simulink subsystem "Vision_Field_Errors_sub"  (R2023b)
settings: Solver=VariableStepAuto  StartTime=0.0  StopTime=10.0  RelTol=1e-3
undefined symbols (not defined in the file): AT_Cage_L_Finish_Angle_Blue, AT_Cage_L_Finish_Angle_Red, AT_Cage_L_Finish_X_Blue, AT_Cage_L_Finish_X_Red, AT_Cage_L_Finish_Y_Blue, AT_Cage_L_Finish_Y_Red, AT_Cage_L_Start_Angle_Blue, AT_Cage_L_Start_Angle_Red, AT_Cage_L_Start_X_Blue, AT_Cage_L_Start_X_Red, AT_Cage_L_Start_Y_Blue, AT_Cage_L_Start_Y_Red, AT_Cage_M_Finish_Angle_Blue, AT_Cage_M_Finish_Angle_Red, AT_Cage_M_Finish_X_Blue, AT_Cage_M_Finish_X_Red, AT_Cage_M_Finish_Y_Blue, AT_Cage_M_Finish_Y_Red, AT_Cage_M_Start_Angle_Blue, AT_Cage_M_Start_Angle_Red, AT_Cage_M_Start_X_Blue, AT_Cage_M_Start_X_Red, AT_Cage_M_Start_Y_Blue, AT_Cage_M_Start_Y_Red, AT_Cage_R_Finish_Angle_Blue, AT_Cage_R_Finish_Angle_Red, AT_Cage_R_Finish_X_Blue, AT_Cage_R_Finish_X_Red, AT_Cage_R_Finish_Y_Blue, AT_Cage_R_Finish_Y_Red, AT_Cage_R_Start_Angle_Blue, AT_Cage_R_Start_Angle_Red, AT_Cage_R_Start_X_Blue, AT_Cage_R_Start_X_Red, AT_Cage_R_Start_Y_Blue, AT_Cage_R_Start_Y_Red, AT_CS_L_Angle_Blue, AT_CS_L_Angle_Red, AT_CS_L_X_Blue, AT_CS_L_X_Red, AT_CS_L_Y_Blue, AT_CS_L_Y_Red, AT_CS_R_Angle_Blue, AT_CS_R_Angle_Red, AT_CS_R_X_Blue, AT_CS_R_X_Red, AT_CS_R_Y_Blue, AT_CS_R_Y_Red, AT_Processor_Angle_Blue, AT_Processor_Angle_Red, AT_Processor_X_Blue, AT_Processor_X_Red, AT_Processor_Y_Blue, AT_Processor_Y_Red
settings Model: Creator=ander  LastModifiedBy=ander

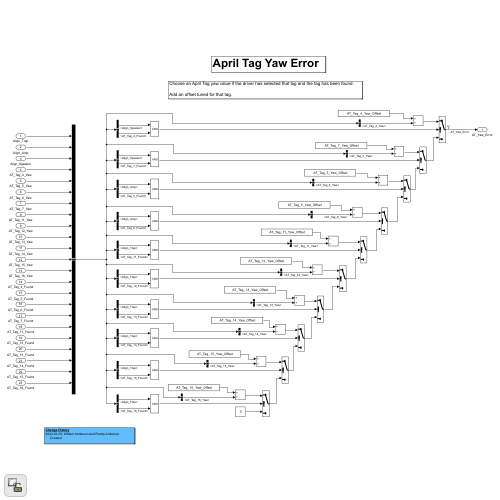
[thumbnail: Simulink's stored preview of the top-level diagram]
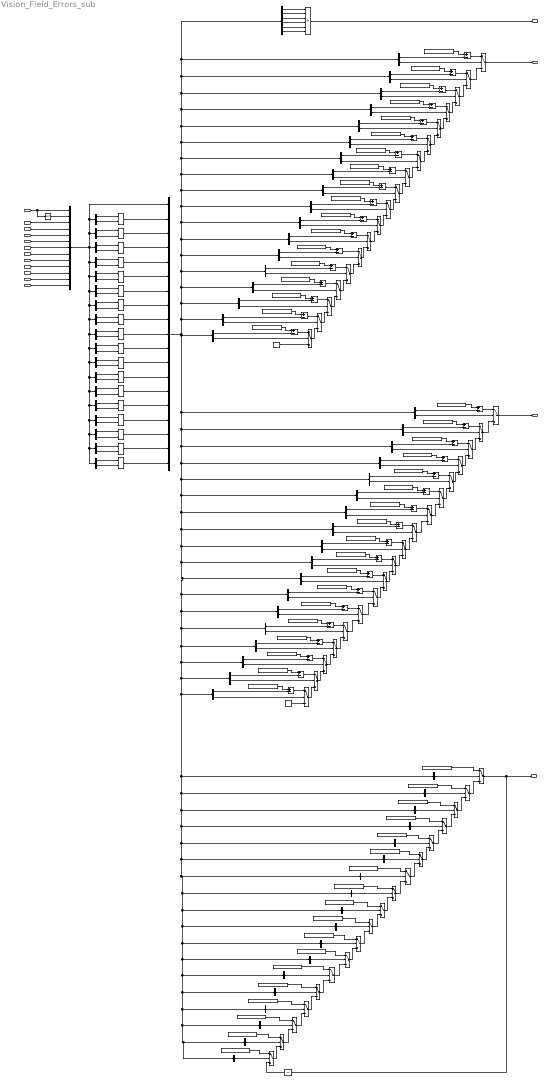
== system Vision_Field_Errors_sub ==
  note: Find an April Tag error value if the driver has selected the tag type and the tag has been found.
      | - Set speaker angle to upstream calculated value.
      | - Set amp and trap angles to known values.
      | - For the x and y errors, calculate the difference relative to the known April tag location.
  note: Change History
      | 2024-03-09, William Anderson and Randy Anderson
      | Created
      | 2024-03-xx, Randy Anderson
      | Various updates to get things working.
  note: April Tag
      | Field Angles and Position Errors
  note: Cage end
  IsBlueAlliance : Inport
  Pose_X : Inport  Port=2
  Pose_Y : Inport  Port=3
  Coral_Station_Left : Inport  Port=4
  Coral_Station_Right : Inport  Port=5
  Processor : Inport  Port=6
  Cage_Left_Start : Inport  Port=7
  Cage_Middle_Start : Inport  Port=8
  Cage_Right_Start : Inport  Port=9
  Cage_Left_Finish : Inport  Port=10
  Cage_Middle_Finish : Inport  Port=11
  Cage_Right_Finish : Inport  Port=12
  Add{1..36} (36 alike) : Sum  Inputs=+-
  Bus Creator : BusCreator  Inputs=13
  Bus Creator1 : BusCreator  Inputs=19
  Bus Selector1 : BusSelector  OutputSignals=Coral_Station_Left,IsBlueAlliance
  Bus Selector10 : BusSelector  OutputSignals=Processor,IsRedAlliance
  Bus Selector11 : BusSelector  OutputSignals=AT_CS_Right_Red_Active
  Bus Selector12 : BusSelector  OutputSignals=Cage_Right_Start,IsRedAlliance
  Bus Selector13 : BusSelector  OutputSignals=AT_Processor_Blue_Active
  Bus Selector14 : BusSelector  OutputSignals=Cage_Middle_Start,IsBlueAlliance
  Bus Selector15 : BusSelector  OutputSignals=AT_Processor_Red_Active
  Bus Selector16 : BusSelector  OutputSignals=Cage_Middle_Start,IsRedAlliance
  Bus Selector17 : BusSelector  OutputSignals=Inputs.Pose_X,AT_Cage_Left_Start_Blue_Active
  Bus Selector18 : BusSelector  OutputSignals=Cage_Left_Start,IsRedAlliance
  Bus Selector19 : BusSelector  OutputSignals=Inputs.Pose_X,AT_Cage_Left_Start_Red_Active
  Bus Selector2 : BusSelector  OutputSignals=Coral_Station_Right,IsBlueAlliance
  Bus Selector20 : BusSelector  OutputSignals=Inputs.Pose_X,AT_CS_Right_Blue_Active
  Bus Selector21 : BusSelector  OutputSignals=Inputs.Pose_Y,AT_CS_Right_Blue_Active
  Bus Selector22 : BusSelector  OutputSignals=Inputs.Pose_Y,AT_CS_Right_Red_Active
  Bus Selector23 : BusSelector  OutputSignals=Inputs.Pose_X,AT_CS_Right_Red_Active
  Bus Selector24 : BusSelector  OutputSignals=Inputs.Pose_X,AT_Processor_Blue_Active
  Bus Selector25 : BusSelector  OutputSignals=Inputs.Pose_X,AT_Processor_Red_Active
  Bus Selector26 : BusSelector  OutputSignals=Inputs.Pose_X,AT_Cage_Middle_Start_Blue_Active
  Bus Selector27 : BusSelector  OutputSignals=Inputs.Pose_X,AT_CS_Left_Blue_Active
  Bus Selector28 : BusSelector  OutputSignals=Inputs.Pose_X,AT_CS_Left_Red_Active
  Bus Selector29 : BusSelector  OutputSignals=Inputs.Pose_X,AT_Cage_Middle_Start_Red_Active
  Bus Selector3 : BusSelector  OutputSignals=Cage_Left_Start,IsBlueAlliance
  Bus Selector30 : BusSelector  OutputSignals=Inputs.Pose_Y,AT_Processor_Blue_Active
  Bus Selector31 : BusSelector  OutputSignals=Inputs.Pose_Y,AT_Processor_Red_Active
  Bus Selector32 : BusSelector  OutputSignals=Inputs.Pose_X,AT_Cage_Right_Start_Blue_Active
  Bus Selector33 : BusSelector  OutputSignals=Inputs.Pose_Y,AT_CS_Left_Blue_Active
  Bus Selector34 : BusSelector  OutputSignals=Inputs.Pose_Y,AT_CS_Left_Red_Active
  Bus Selector35 : BusSelector  OutputSignals=Inputs.Pose_X,AT_Cage_Right_Start_Red_Active
  Bus Selector36 : BusSelector  OutputSignals=Inputs.Coral_Station_Left,Inputs.Coral_Station_Right,Inputs.Processor,Inputs.Cage_Left_Start,Inputs.Cage_Middle_Start,Inputs.Cage_Right_Start
  Bus Selector37 : BusSelector  OutputSignals=Cage_Right_Start,IsBlueAlliance
  Bus Selector38 : BusSelector  OutputSignals=Cage_Right_Finish,IsRedAlliance
  Bus Selector39 : BusSelector  OutputSignals=Cage_Middle_Finish,IsBlueAlliance
  Bus Selector4 : BusSelector  OutputSignals=Coral_Station_Right,IsRedAlliance
  Bus Selector40 : BusSelector  OutputSignals=Cage_Middle_Finish,IsRedAlliance
  Bus Selector41 : BusSelector  OutputSignals=Cage_Left_Finish,IsRedAlliance
  Bus Selector42 : BusSelector  OutputSignals=Cage_Left_Finish,IsBlueAlliance
  Bus Selector43 : BusSelector  OutputSignals=Cage_Right_Finish,IsBlueAlliance
  Bus Selector44 : BusSelector  OutputSignals=Inputs.Pose_Y,AT_Cage_Middle_Start_Blue_Active
  Bus Selector45 : BusSelector  OutputSignals=Inputs.Pose_Y,AT_Cage_Middle_Start_Red_Active
  Bus Selector46 : BusSelector  OutputSignals=Inputs.Pose_Y,AT_Cage_Right_Start_Blue_Active
  Bus Selector47 : BusSelector  OutputSignals=Inputs.Pose_Y,AT_Cage_Right_Start_Red_Active
  Bus Selector48 : BusSelector  OutputSignals=Inputs.Pose_Y,AT_Cage_Left_Start_Blue_Active
  Bus Selector49 : BusSelector  OutputSignals=Inputs.Pose_Y,AT_Cage_Left_Start_Red_Active
  Bus Selector5 : BusSelector  OutputSignals=AT_CS_Left_Blue_Active
  Bus Selector50 : BusSelector  OutputSignals=Inputs.Pose_X,AT_Cage_Left_Finish_Blue_Active
  Bus Selector51 : BusSelector  OutputSignals=Inputs.Pose_X,AT_Cage_Left_Finish_Red_Active
  Bus Selector52 : BusSelector  OutputSignals=Inputs.Pose_X,AT_Cage_Middle_Finish_Blue_Active
  Bus Selector53 : BusSelector  OutputSignals=Inputs.Pose_X,AT_Cage_Middle_Finish_Red_Active
  Bus Selector54 : BusSelector  OutputSignals=Inputs.Pose_X,AT_Cage_Right_Finish_Blue_Active
  Bus Selector55 : BusSelector  OutputSignals=Inputs.Pose_X,AT_Cage_Right_Finish_Red_Active
  Bus Selector56 : BusSelector  OutputSignals=Inputs.Pose_Y,AT_Cage_Middle_Finish_Blue_Active
  Bus Selector57 : BusSelector  OutputSignals=Inputs.Pose_Y,AT_Cage_Middle_Finish_Red_Active
  Bus Selector58 : BusSelector  OutputSignals=Inputs.Pose_Y,AT_Cage_Right_Finish_Blue_Active
  Bus Selector59 : BusSelector  OutputSignals=Inputs.Pose_Y,AT_Cage_Right_Finish_Red_Active
  Bus Selector6 : BusSelector  OutputSignals=Coral_Station_Left,IsRedAlliance
  Bus Selector60 : BusSelector  OutputSignals=Inputs.Pose_Y,AT_Cage_Left_Finish_Blue_Active
  Bus Selector61 : BusSelector  OutputSignals=Inputs.Pose_Y,AT_Cage_Left_Finish_Red_Active
  Bus Selector62 : BusSelector  OutputSignals=AT_Cage_Middle_Start_Red_Active
  Bus Selector63 : BusSelector  OutputSignals=AT_Cage_Right_Start_Blue_Active
  Bus Selector64 : BusSelector  OutputSignals=AT_Cage_Right_Start_Red_Active
  Bus Selector65 : BusSelector  OutputSignals=AT_Cage_Left_Start_Blue_Active
  Bus Selector66 : BusSelector  OutputSignals=AT_Cage_Left_Start_Red_Active
  Bus Selector67 : BusSelector  OutputSignals=AT_Cage_Middle_Start_Blue_Active
  Bus Selector68 : BusSelector  OutputSignals=AT_Cage_Middle_Finish_Red_Active
  Bus Selector69 : BusSelector  OutputSignals=AT_Cage_Right_Finish_Blue_Active
  Bus Selector7 : BusSelector  OutputSignals=AT_CS_Left_Red_Active
  Bus Selector70 : BusSelector  OutputSignals=AT_Cage_Right_Finish_Red_Active
  Bus Selector71 : BusSelector  OutputSignals=AT_Cage_Left_Finish_Blue_Active
  Bus Selector72 : BusSelector  OutputSignals=AT_Cage_Left_Finish_Red_Active
  Bus Selector73 : BusSelector  OutputSignals=AT_Cage_Middle_Finish_Blue_Active
  Bus Selector8 : BusSelector  OutputSignals=Processor,IsBlueAlliance
  Bus Selector9 : BusSelector  OutputSignals=AT_CS_Right_Blue_Active
  Constant1 : Constant  Value=AT_Cage_R_Start_Angle_Blue
  Constant10 : Constant  Value=AT_Processor_Angle_Blue
  Constant11 : Constant  Value=AT_CS_R_Angle_Red
  Constant12 : Constant  Value=AT_CS_R_Angle_Blue
  Constant13 : Constant  Value=AT_CS_L_Angle_Red
  Constant14 : Constant  Value=AT_CS_L_Angle_Blue
  Constant15 : Constant  Value=AT_Cage_L_Start_X_Red
  Constant16 : Constant  Value=AT_Cage_R_Start_Y_Red
  Constant17 : Constant  Value=AT_CS_R_X_Red
  Constant18 : Constant  Value=AT_Processor_X_Blue
  Constant19 : Constant  Value=AT_Processor_X_Red
  Constant2 : Constant  Value=AT_Cage_L_Finish_X_Red
  Constant20 : Constant  Value=AT_Cage_M_Start_X_Blue
  Constant21 : Constant  Value=AT_Processor_Y_Blue
  Constant22 : Constant  Value=AT_Cage_M_Start_Y_Blue
  Constant23 : Constant  Value=AT_Processor_Y_Red
  Constant24 : Constant  Value=AT_Cage_M_Start_X_Red
  Constant25 : Constant  Value=AT_Cage_L_Start_Y_Red
  Constant26 : Constant  Value=AT_CS_R_Y_Blue
  Constant27 : Constant  Value=AT_CS_L_Y_Red
  Constant28 : Constant  Value=AT_CS_L_Y_Blue
  Constant29 : Constant  Value=AT_Cage_R_Start_X_Blue
  Constant3 : Constant  Value=AT_CS_R_Y_Red
  Constant30 : Constant  Value=0
  Constant31 : Constant  Value=AT_Cage_R_Start_X_Red
  Constant32 : Constant  Value=AT_Cage_L_Start_Y_Blue
  Constant33 : Constant  Value=AT_Cage_M_Start_Y_Red
  Constant34 : Constant  Value=AT_Cage_M_Finish_X_Blue
  Constant35 : Constant  Value=AT_Cage_M_Finish_X_Red
  Constant36 : Constant  Value=AT_Cage_R_Finish_X_Blue
  Constant37 : Constant  Value=0
  Constant38 : Constant  Value=AT_Cage_R_Finish_X_Red
  Constant39 : Constant  Value=AT_Cage_L_Finish_X_Blue
  Constant4 : Constant  Value=AT_CS_R_X_Blue
  Constant40 : Constant  Value=AT_Cage_R_Finish_Y_Red
  Constant41 : Constant  Value=AT_Cage_M_Finish_Y_Blue
  Constant42 : Constant  Value=AT_Cage_L_Finish_Y_Red
  Constant43 : Constant  Value=AT_Cage_L_Finish_Y_Blue
  Constant44 : Constant  Value=AT_Cage_M_Finish_Y_Red
  Constant45 : Constant  Value=AT_Cage_R_Finish_Y_Blue
  Constant46 : Constant  Value=AT_Cage_M_Start_Angle_Red
  Constant47 : Constant  Value=AT_Cage_M_Start_Angle_Blue
  Constant48 : Constant  Value=AT_Cage_L_Start_Angle_Red
  Constant49 : Constant  Value=AT_Cage_L_Start_Angle_Blue
  Constant5 : Constant  Value=AT_CS_L_X_Red
  Constant50 : Constant  Value=AT_Cage_R_Start_Angle_Red
  Constant51 : Constant  Value=AT_Cage_R_Finish_Angle_Blue
  Constant52 : Constant  Value=AT_Cage_M_Finish_Angle_Red
  Constant53 : Constant  Value=AT_Cage_M_Finish_Angle_Blue
  Constant54 : Constant  Value=AT_Cage_L_Finish_Angle_Red
  Constant55 : Constant  Value=AT_Cage_L_Finish_Angle_Blue
  Constant56 : Constant  Value=AT_Cage_R_Finish_Angle_Red
  Constant6 : Constant  Value=AT_Cage_R_Start_Y_Blue
  Constant7 : Constant  Value=AT_Cage_L_Start_X_Blue
  Constant8 : Constant  Value=AT_Processor_Angle_Red
  Constant9 : Constant  Value=AT_CS_L_X_Blue
  Logical Operator{1..9,12..20} (18 alike) : Logic  AllPortsSameDT=off  OutDataTypeStr=boolean
  Logical Operator10 : Logic  Operator=NOT  AllPortsSameDT=off  OutDataTypeStr=boolean
  Logical Operator11 : Logic  Operator=OR  Inputs=6  AllPortsSameDT=off  OutDataTypeStr=boolean
  Switch{1..54} (54 alike) : Switch  Criteria=u2 ~= 0  SaturateOnIntegerOverflow=off  InputSameDT=off
  Unit Delay1 : UnitDelay  SampleTime=-1  HasFrameUpgradeWarning=on
  AT_Field_Enable : Outport
  AT_Field_Error_X : Outport  Port=2
  AT_Field_Error_Y : Outport  Port=3
  AT_Field_Target_Angle : Outport  Port=4
  wires:
  Bus Selector15/1 -> Switch9/2  "<AT_Processor_Red_Active>"
  Bus Selector38/1 -> Logical Operator17/1  "<Cage_Right_Finish>"
  Bus Selector40/1 -> Logical Operator15/1  "<Cage_Middle_Finish>"
  Bus Selector40/2 -> Logical Operator15/2  "<IsRedAlliance>"
  Bus Selector41/1 -> Logical Operator20/1  "<Cage_Left_Finish>"
  Logical Operator15/1 -> Bus Creator1/17  "AT_Cage_Middle_Finish_Red_Active"
  Bus Selector38/2 -> Logical Operator17/2  "<IsRedAlliance>"
  Bus Selector39/2 -> Logical Operator18/2  "<IsBlueAlliance>"
  Logical Operator19/1 -> Bus Creator1/14  "AT_Cage_Left_Finish_Blue_Active"
  Logical Operator20/1 -> Bus Creator1/15  "AT_Cage_Left_Finish_Red_Active"
  Logical Operator18/1 -> Bus Creator1/16  "AT_Cage_Middle_Finish_Blue_Active"
  Logical Operator17/1 -> Bus Creator1/19  "AT_Cage_Right_Finish_Red_Active"
  Bus Selector41/2 -> Logical Operator20/2  "<IsRedAlliance>"
  Logical Operator16/1 -> Bus Creator1/18  "AT_Cage_Right_Finish_Blue_Active"
  Bus Selector43/1 -> Logical Operator16/1  "<Cage_Right_Finish>"
  Bus Selector42/1 -> Logical Operator19/1  "<Cage_Left_Finish>"
  Bus Selector42/2 -> Logical Operator19/2  "<IsBlueAlliance>"
  Bus Selector39/1 -> Logical Operator18/1  "<Cage_Middle_Finish>"
  Bus Selector43/2 -> Logical Operator16/2  "<IsBlueAlliance>"
  Cage_Left_Finish/1 -> Bus Creator/11
  Cage_Middle_Finish/1 -> Bus Creator/12
  Cage_Right_Finish/1 -> Bus Creator/13
  Switch15/1 -> Unit Delay1/1, AT_Field_Target_Angle/1  "AT_Field_Target_Angle"
  Switch4/1 -> AT_Field_Error_Y/1  "AT_Field_Error_Y"
  Switch2/1 -> AT_Field_Error_X/1  "AT_Field_Error_X"
  Logical Operator14/1 -> Bus Creator1/13  "AT_Cage_Right_Start_Red_Active"
  Logical Operator13/1 -> Bus Creator1/12  "AT_Cage_Right_Start_Blue_Active"
  Logical Operator12/1 -> Bus Creator1/11  "AT_Cage_Middle_Start_Red_Active"
  Logical Operator7/1 -> Bus Creator1/10  "AT_Cage_Middle_Start_Blue_Active"
  Logical Operator9/1 -> Bus Creator1/9  "AT_Cage_Left_Start_Red_Active"
  Logical Operator8/1 -> Bus Creator1/8  "AT_Cage_Left_Start_Blue_Active"
  Bus Selector36/6 -> Logical Operator11/6  "<Cage_Right_Start>"
  Bus Selector36/5 -> Logical Operator11/5  "<Cage_Middle_Start>"
  Bus Selector36/4 -> Logical Operator11/4  "<Cage_Left_Start>"
  Bus Selector37/1 -> Logical Operator13/1  "<Cage_Right_Start>"
  Bus Selector37/2 -> Logical Operator13/2  "<IsBlueAlliance>"
  Bus Selector14/1 -> Logical Operator7/1  "<Cage_Middle_Start>"
  Bus Selector12/2 -> Logical Operator14/2  "<IsRedAlliance>"
  Bus Selector12/1 -> Logical Operator14/1  "<Cage_Right_Start>"
  Bus Selector18/2 -> Logical Operator9/2  "<IsRedAlliance>"
  Bus Selector18/1 -> Logical Operator9/1  "<Cage_Left_Start>"
  Bus Selector3/1 -> Logical Operator8/1  "<Cage_Left_Start>"
  Bus Selector3/2 -> Logical Operator8/2  "<IsBlueAlliance>"
  Bus Selector16/1 -> Logical Operator12/1  "<Cage_Middle_Start>"
  Bus Selector16/2 -> Logical Operator12/2  "<IsRedAlliance>"
  Bus Selector14/2 -> Logical Operator7/2  "<IsBlueAlliance>"
  Cage_Right_Start/1 -> Bus Creator/10
  Cage_Middle_Start/1 -> Bus Creator/9
  Cage_Left_Start/1 -> Bus Creator/8
  Logical Operator6/1 -> Bus Creator1/7  "AT_Processor_Red_Active"
  Logical Operator5/1 -> Bus Creator1/6  "AT_Processor_Blue_Active"
  Bus Selector10/1 -> Logical Operator6/1  "<Processor>"
  Bus Selector8/2 -> Logical Operator5/2  "<IsBlueAlliance>"
  Bus Selector10/2 -> Logical Operator6/2  "<IsRedAlliance>"
  Bus Selector8/1 -> Logical Operator5/1  "<Processor>"
  Logical Operator4/1 -> Bus Creator1/5  "AT_CS_Right_Red_Active"
  Logical Operator1/1 -> Bus Creator1/4  "AT_CS_Right_Blue_Active"
  Bus Selector4/1 -> Logical Operator4/1  "<Coral_Station_Right>"
  Bus Selector2/1 -> Logical Operator1/1  "<Coral_Station_Right>"
  Bus Selector2/2 -> Logical Operator1/2  "<IsBlueAlliance>"
  Bus Selector4/2 -> Logical Operator4/2  "<IsRedAlliance>"
  Processor/1 -> Bus Creator/7
  Coral_Station_Right/1 -> Bus Creator/6
  Coral_Station_Left/1 -> Bus Creator/5
  Pose_Y/1 -> Bus Creator/4
  Pose_X/1 -> Bus Creator/3
  Logical Operator10/1 -> Bus Creator/2  "IsRedAlliance"
  Logical Operator11/1 -> AT_Field_Enable/1  "AT_Field_Enable"
  Bus Selector36/3 -> Logical Operator11/3  "<Processor>"
  Bus Selector36/2 -> Logical Operator11/2  "<Coral_Station_Right>"
  Bus Selector36/1 -> Logical Operator11/1  "<Coral_Station_Left>"
  Constant8/1 -> Switch9/1
  Constant10/1 -> Switch8/1
  Constant11/1 -> Switch7/1
  Constant12/1 -> Switch6/1
  Constant13/1 -> Switch5/1
  Constant14/1 -> Switch15/1
  Bus Selector6/2 -> Logical Operator3/2  "<IsRedAlliance>"
  Bus Selector1/2 -> Logical Operator2/2  "<IsBlueAlliance>"
  IsBlueAlliance/1 -> Logical Operator10/1, Bus Creator/1
  Constant5/1 -> Add16/1
  Add16/1 -> Switch16/1
  Add17/1 -> Switch2/1
  Constant9/1 -> Add17/1
  Switch16/1 -> Switch2/3
  Bus Selector13/1 -> Switch8/2  "<AT_Processor_Blue_Active>"
  Bus Selector11/1 -> Switch7/2  "<AT_CS_Right_Red_Active>"
  Bus Selector9/1 -> Switch6/2  "<AT_CS_Right_Blue_Active>"
  Bus Selector7/1 -> Switch5/2  "<AT_CS_Left_Red_Active>"
  Bus Selector5/1 -> Switch15/2  "<AT_CS_Left_Blue_Active>"
  Logical Operator3/1 -> Bus Creator1/3  "AT_CS_Left_Red_Active"
  Logical Operator2/1 -> Bus Creator1/2  "AT_CS_Left_Blue_Active"
  Bus Selector1/1 -> Logical Operator2/1  "<Coral_Station_Left>"
  Switch7/1 -> Switch6/3
  Switch5/1 -> Switch15/3
  Bus Selector6/1 -> Logical Operator3/1  "<Coral_Station_Left>"
  Switch6/1 -> Switch5/3
  Switch9/1 -> Switch8/3
  Bus Creator/1 -> Bus Creator1/1, Bus Selector1/1, Bus Selector6/1, Bus Selector4/1, Bus Selector8/1, Bus Selector38/1, Bus Selector43/1, Bus Selector40/1, Bus Selector39/1, Bus Selector41/1, Bus Selector42/1, Bus Selector12/1, Bus Selector37/1, Bus Selector16/1, Bus Selector14/1, Bus Selector18/1, Bus Selector3/1, Bus Selector10/1, Bus Selector2/1  "Inputs"
  Switch8/1 -> Switch7/3
  Bus Selector27/1 -> Add17/2  "<Pose_X>"
  Bus Selector27/2 -> Switch2/2  "<AT_CS_Left_Blue_Active>"
  Bus Selector28/1 -> Add16/2  "<Pose_X>"
  Bus Selector28/2 -> Switch16/2  "<AT_CS_Left_Red_Active>"
  Bus Selector20/2 -> Switch1/2  "<AT_CS_Right_Blue_Active>"
  Bus Selector20/1 -> Add10/2  "<Pose_X>"
  Add10/1 -> Switch1/1
  Constant4/1 -> Add10/1
  Bus Selector23/2 -> Switch12/2  "<AT_CS_Right_Red_Active>"
  Bus Selector23/1 -> Add11/2  "<Pose_X>"
  Add11/1 -> Switch12/1
  Constant17/1 -> Add11/1
  Constant18/1 -> Add14/1
  Bus Selector24/1 -> Add14/2  "<Pose_X>"
  Bus Selector24/2 -> Switch13/2  "<AT_Processor_Blue_Active>"
  Add14/1 -> Switch13/1
  Constant19/1 -> Add15/1
  Bus Selector25/1 -> Add15/2  "<Pose_X>"
  Bus Selector25/2 -> Switch14/2  "<AT_Processor_Red_Active>"
  Add15/1 -> Switch14/1
  Switch1/1 -> Switch16/3
  Switch12/1 -> Switch1/3
  Switch13/1 -> Switch12/3
  Switch14/1 -> Switch13/3
  Bus Selector31/1 -> Add21/2  "<Pose_Y>"
  Constant26/1 -> Add12/1
  Add12/1 -> Switch19/1
  Switch19/1 -> Switch24/3
  Bus Selector21/2 -> Switch19/2  "<AT_CS_Right_Blue_Active>"
  Add20/1 -> Switch21/1
  Bus Selector30/2 -> Switch21/2  "<AT_Processor_Blue_Active>"
  Bus Selector21/1 -> Add12/2  "<Pose_Y>"
  Constant23/1 -> Add21/1
  Switch20/1 -> Switch19/3
  Bus Selector31/2 -> Switch22/2  "<AT_Processor_Red_Active>"
  Constant3/1 -> Add13/1
  Add13/1 -> Switch20/1
  Switch21/1 -> Switch20/3
  Add21/1 -> Switch22/1
  Bus Selector34/2 -> Switch24/2  "<AT_CS_Left_Red_Active>"
  Bus Selector33/2 -> Switch4/2  "<AT_CS_Left_Blue_Active>"
  Bus Selector22/2 -> Switch20/2  "<AT_CS_Right_Red_Active>"
  Switch22/1 -> Switch21/3
  Bus Selector34/1 -> Add22/2  "<Pose_Y>"
  Bus Selector33/1 -> Add23/2  "<Pose_Y>"
  Constant21/1 -> Add20/1
  Switch24/1 -> Switch4/3
  Bus Selector22/1 -> Add13/2  "<Pose_Y>"
  Add23/1 -> Switch4/1
  Bus Selector30/1 -> Add20/2  "<Pose_Y>"
  Add22/1 -> Switch24/1
  Constant28/1 -> Add23/1
  Constant27/1 -> Add22/1
  Switch3/1 -> Switch14/3
  Bus Selector17/2 -> Switch3/2  "<AT_Cage_Left_Start_Blue_Active>"
  Add1/1 -> Switch3/1
  Constant7/1 -> Add1/1
  Bus Selector17/1 -> Add1/2  "<Pose_X>"
  Switch10/1 -> Switch3/3
  Bus Selector19/2 -> Switch10/2  "<AT_Cage_Left_Start_Red_Active>"
  Add2/1 -> Switch10/1
  Constant15/1 -> Add2/1
  Bus Selector19/1 -> Add2/2  "<Pose_X>"
  Switch11/1 -> Switch10/3
  Bus Selector26/2 -> Switch11/2  "<AT_Cage_Middle_Start_Blue_Active>"
  Add3/1 -> Switch11/1
  Constant20/1 -> Add3/1
  Bus Selector26/1 -> Add3/2  "<Pose_X>"
  Switch17/1 -> Switch11/3
  Bus Selector29/2 -> Switch17/2  "<AT_Cage_Middle_Start_Red_Active>"
  Add4/1 -> Switch17/1
  Constant24/1 -> Add4/1
  Bus Selector29/1 -> Add4/2  "<Pose_X>"
  Switch18/1 -> Switch17/3
  Bus Selector32/2 -> Switch18/2  "<AT_Cage_Right_Start_Blue_Active>"
  Add5/1 -> Switch18/1
  Constant29/1 -> Add5/1
  Bus Selector32/1 -> Add5/2  "<Pose_X>"
  Switch23/1 -> Switch18/3
  Bus Selector35/2 -> Switch23/2  "<AT_Cage_Right_Start_Red_Active>"
  Add6/1 -> Switch23/1
  Constant31/1 -> Add6/1
  Bus Selector35/1 -> Add6/2  "<Pose_X>"
  Bus Selector46/1 -> Add9/2  "<Pose_Y>"
  Constant16/1 -> Add18/1
  Bus Selector49/2 -> Switch29/2  "<AT_Cage_Left_Start_Red_Active>"
  Add24/1 -> Switch30/1
  Switch29/1 -> Switch30/3
  Bus Selector48/2 -> Switch30/2  "<AT_Cage_Left_Start_Blue_Active>"
  Switch28/1 -> Switch27/3
  Add8/1 -> Switch26/1
  Switch25/1 -> Switch29/3
  Bus Selector47/2 -> Switch28/2  "<AT_Cage_Right_Start_Red_Active>"
  Constant33/1 -> Add8/1
  Bus Selector45/2 -> Switch26/2  "<AT_Cage_Middle_Start_Red_Active>"
  Add9/1 -> Switch27/1
  Bus Selector44/2 -> Switch25/2  "<AT_Cage_Middle_Start_Blue_Active>"
  Switch27/1 -> Switch26/3
  Constant25/1 -> Add19/1
  Constant32/1 -> Add24/1
  Add7/1 -> Switch25/1
  Bus Selector44/1 -> Add7/2  "<Pose_Y>"
  Bus Selector48/1 -> Add24/2  "<Pose_Y>"
  Bus Selector49/1 -> Add19/2  "<Pose_Y>"
  Bus Selector45/1 -> Add8/2  "<Pose_Y>"
  Add19/1 -> Switch29/1
  Constant22/1 -> Add7/1
  Add18/1 -> Switch28/1
  Switch26/1 -> Switch25/3
  Bus Selector46/2 -> Switch27/2  "<AT_Cage_Right_Start_Blue_Active>"
  Bus Selector47/1 -> Add18/2  "<Pose_Y>"
  Constant6/1 -> Add9/1
  Switch30/1 -> Switch22/3
  Add30/1 -> Switch35/1
  Bus Selector55/2 -> Switch35/2  "<AT_Cage_Right_Finish_Red_Active>"
  Bus Selector55/1 -> Add30/2  "<Pose_X>"
  Switch35/1 -> Switch34/3
  Constant38/1 -> Add30/1
  Constant37/1 -> Switch35/3
  Switch33/1 -> Switch32/3
  Add29/1 -> Switch34/1
  Bus Selector54/2 -> Switch34/2  "<AT_Cage_Right_Finish_Blue_Active>"
  Switch36/1 -> Switch23/3
  Bus Selector54/1 -> Add29/2  "<Pose_X>"
  Switch34/1 -> Switch33/3
  Constant39/1 -> Add25/1
  Switch31/1 -> Switch36/3
  Constant36/1 -> Add29/1
  Switch32/1 -> Switch31/3
  Bus Selector50/2 -> Switch36/2  "<AT_Cage_Left_Finish_Blue_Active>"
  Bus Selector51/1 -> Add26/2  "<Pose_X>"
  Add26/1 -> Switch31/1
  Constant2/1 -> Add26/1
  Bus Selector51/2 -> Switch31/2  "<AT_Cage_Left_Finish_Red_Active>"
  Bus Selector53/1 -> Add28/2  "<Pose_X>"
  Add28/1 -> Switch33/1
  Constant35/1 -> Add28/1
  Bus Selector53/2 -> Switch33/2  "<AT_Cage_Middle_Finish_Red_Active>"
  Constant34/1 -> Add27/1
  Bus Selector52/2 -> Switch32/2  "<AT_Cage_Middle_Finish_Blue_Active>"
  Bus Selector52/1 -> Add27/2  "<Pose_X>"
  Add25/1 -> Switch36/1
  Add27/1 -> Switch32/1
  Bus Selector50/1 -> Add25/2  "<Pose_X>"
  Switch37/1 -> Switch41/3
  Bus Selector59/2 -> Switch40/2  "<AT_Cage_Right_Finish_Red_Active>"
  Bus Selector57/2 -> Switch38/2  "<AT_Cage_Middle_Finish_Red_Active>"
  Bus Selector56/1 -> Add34/2  "<Pose_Y>"
  Switch40/1 -> Switch39/3
  Add34/1 -> Switch37/1
  Bus Creator1/1 -> Bus Selector54/1, Bus Selector53/1, Bus Selector52/1, Bus Selector51/1, Bus Selector50/1, Bus Selector35/1, Bus Selector32/1, Bus Selector29/1, Bus Selector26/1, Bus Selector19/1, Bus Selector17/1, Bus Selector23/1, Bus Selector28/1, Bus Selector36/1, Bus Selector27/1, Bus Selector20/1, Bus Selector24/1, Bus Selector25/1, Bus Selector55/1, Bus Selector33/1, Bus Selector34/1, Bus Selector21/1, Bus Selector22/1, Bus Selector30/1, Bus Selector31/1, Bus Selector47/1, Bus Selector15/1, Bus Selector65/1, Bus Selector66/1, Bus Selector67/1, Bus Selector62/1, Bus Selector63/1, Bus Selector64/1, Bus Selector71/1, Bus Selector70/1, Bus Selector69/1, Bus Selector68/1, Bus Selector73/1, Bus Selector72/1, Bus Selector13/1, Bus Selector11/1, Bus Selector9/1, Bus Selector7/1, Bus Selector5/1, Bus Selector59/1, Bus Selector58/1, Bus Selector57/1, Bus Selector56/1, Bus Selector61/1, Bus Selector60/1, Bus Selector46/1, Bus Selector45/1, Bus Selector44/1, Bus Selector49/1, Bus Selector48/1
  Constant45/1 -> Add36/1
  Bus Selector59/1 -> Add31/2  "<Pose_Y>"
  Bus Selector58/2 -> Switch39/2  "<AT_Cage_Right_Finish_Blue_Active>"
  Bus Selector61/1 -> Add32/2  "<Pose_Y>"
  Add31/1 -> Switch40/1
  Switch42/1 -> Switch28/3
  Constant41/1 -> Add34/1
  Constant44/1 -> Add35/1
  Bus Selector60/1 -> Add33/2  "<Pose_Y>"
  Add32/1 -> Switch41/1
  Bus Selector61/2 -> Switch41/2  "<AT_Cage_Left_Finish_Red_Active>"
  Constant40/1 -> Add31/1
  Add35/1 -> Switch38/1
  Bus Selector58/1 -> Add36/2  "<Pose_Y>"
  Bus Selector57/1 -> Add35/2  "<Pose_Y>"
  Constant43/1 -> Add33/1
  Switch39/1 -> Switch38/3
  Bus Selector56/2 -> Switch37/2  "<AT_Cage_Middle_Finish_Blue_Active>"
  Constant42/1 -> Add32/1
  Constant30/1 -> Switch40/3
  Switch41/1 -> Switch42/3
  Switch38/1 -> Switch37/3
  Bus Selector60/2 -> Switch42/2  "<AT_Cage_Left_Finish_Blue_Active>"
  Add33/1 -> Switch42/1
  Add36/1 -> Switch39/1
  Bus Selector64/1 -> Switch48/2  "<AT_Cage_Right_Start_Red_Active>"
  Switch48/1 -> Switch47/3
  Switch47/1 -> Switch46/3
  Bus Selector66/1 -> Switch44/2  "<AT_Cage_Left_Start_Red_Active>"
  Bus Selector62/1 -> Switch46/2  "<AT_Cage_Middle_Start_Red_Active>"
  Constant46/1 -> Switch46/1
  Constant50/1 -> Switch48/1
  Constant47/1 -> Switch45/1
  Constant1/1 -> Switch47/1
  Constant49/1 -> Switch43/1
  Bus Selector63/1 -> Switch47/2  "<AT_Cage_Right_Start_Blue_Active>"
  Bus Selector67/1 -> Switch45/2  "<AT_Cage_Middle_Start_Blue_Active>"
  Bus Selector65/1 -> Switch43/2  "<AT_Cage_Left_Start_Blue_Active>"
  Switch46/1 -> Switch45/3
  Switch44/1 -> Switch43/3
  Switch45/1 -> Switch44/3
  Constant48/1 -> Switch44/1
  Switch43/1 -> Switch9/3
  Bus Selector70/1 -> Switch54/2  "<AT_Cage_Right_Finish_Red_Active>"
  Switch54/1 -> Switch53/3
  Switch53/1 -> Switch52/3
  Bus Selector72/1 -> Switch50/2  "<AT_Cage_Left_Finish_Red_Active>"
  Bus Selector68/1 -> Switch52/2  "<AT_Cage_Middle_Finish_Red_Active>"
  Constant52/1 -> Switch52/1
  Constant56/1 -> Switch54/1
  Constant53/1 -> Switch51/1
  Constant51/1 -> Switch53/1
  Constant55/1 -> Switch49/1
  Bus Selector69/1 -> Switch53/2  "<AT_Cage_Right_Finish_Blue_Active>"
  Bus Selector73/1 -> Switch51/2  "<AT_Cage_Middle_Finish_Blue_Active>"
  Bus Selector71/1 -> Switch49/2  "<AT_Cage_Left_Finish_Blue_Active>"
  Switch52/1 -> Switch51/3
  Switch50/1 -> Switch49/3
  Switch51/1 -> Switch50/3
  Constant54/1 -> Switch50/1
  Switch49/1 -> Switch48/3
  Unit Delay1/1 -> Switch54/3
